simulink model "Efeitos_da_Amostragem"  (R2025a)
settings: Solver=VariableStepAuto  StartTime=0.0  StopTime=inf  MaxStep=1e-5  RelTol=1e-3
libraries: dspsnks4 x1
settings Model: Creator=rcard  LastModifiedBy=cardo
settings OptimizationCC: ReuseModelBlockBuffer=off
settings RTWCC: GPUComputeCapability=3.5

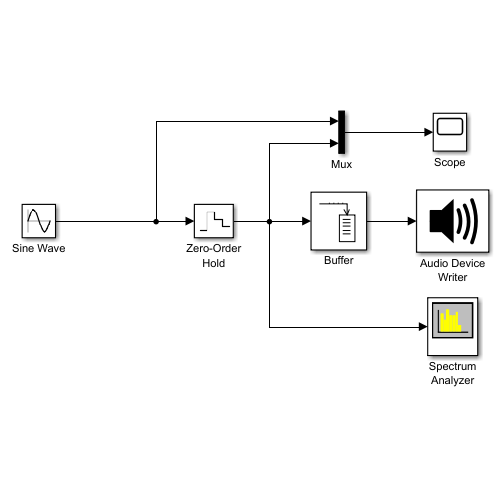
[thumbnail: Simulink's stored preview of the top-level diagram]
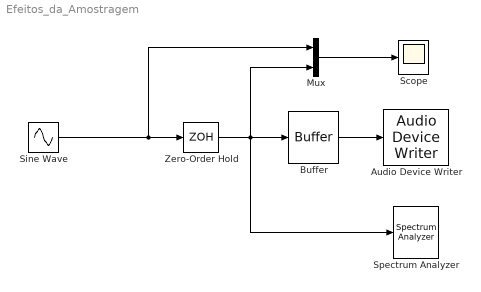
== system Efeitos_da_Amostragem ==
  Audio Device Writer : dspsnks4/Audio Device Writer  Driver=DirectSound  Device=Default  InheritSampleRate=on  SampleRate=44100  BitDepth=24-bit integer  BufferSize=4096  NumBuffers=10  DefaultOutputChannelMapping=on  OutputChannelMapping=1:2  OutputNumUnderrunSamples=off  DriverIdx=1  DeviceWarnFlag=''
  Buffer : Buffer  N=128  OutputFrames=off
  Mux : Mux  Inputs=2
  Scope : Scope
      settings: ActiveDisplayYMinimum=-1.03542  ActiveDisplayYMaximum=1.02988
  Sine Wave : Sin  Frequency=2*pi*5000  Phase=pi/2  SampleTime=0
  Spectrum Analyzer : SpectrumAnalyzer  WindowPosition=[61.000000,12.000000,1584.000000,936.000000,]  ScopeFrameLocation=window  ViewType=Spectrum and spectrogram  SampleRate=2500  PlotAsTwoSidedSpectrum=off  AxesScaling=Manual  Span=24000  CenterFrequency=12000  StartFrequency=0  StopFrequency=1250  AveragingMethod=Exponential  ReferenceLoad=50  YLimits=[-67.6856 16.8013]  ColorLimits=[-67.6856 16.8013]  SelectedToolstripTab=spectrumAnalyzerToolstrip.spectrumTab  AllowFFTLengthLessThanSamplesPerUpdate=on
  Zero-Order Hold : ZeroOrderHold  SampleTime=1/1500
  wires:
  Zero-Order Hold/1 -> Spectrum Analyzer/1, Mux/2, Buffer/1
  Buffer/1 -> Audio Device Writer/1
  Mux/1 -> Scope/1
  Sine Wave/1 -> Mux/1, Zero-Order Hold/1
